simulink model "TDOF_simulink_v2"  (R2026a)
settings: Solver=VariableStepAuto  StopTime=180  MaxStep=0.001
InitFcn:
  | model_path = fileparts(get_param(bdroot, 'FileName'));
  | parent_path = fileparts(model_path);
  | run(fullfile(parent_path, 'scripts', 'NewInitFcn.m'));
undefined symbols (not defined in the file): chute, data, envP, launch, r
libraries: simulink x5
settings Model: Creator=awint  LastModifiedBy=benjaminbrobst

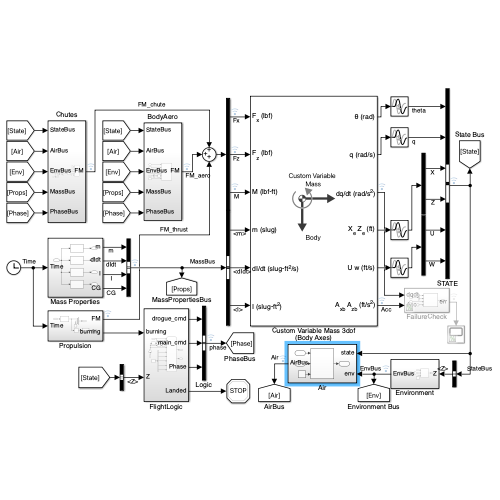
[thumbnail: Simulink's stored preview of the top-level diagram]
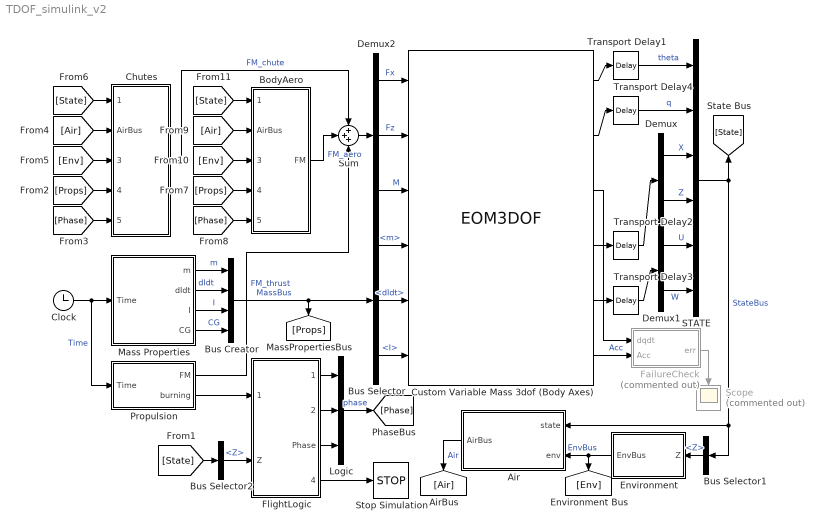
== system TDOF_simulink_v2 ==
  Air : Subsystem
  BodyAero : Subsystem
  Bus Creator : BusCreator  Inputs=4
  Bus Selector : BusSelector  OutputSignals=m,dIdt,I
  Bus Selector1 : BusSelector  OutputSignals=Z
  Bus Selector2 : BusSelector  OutputSignals=Z
  Chutes : Subsystem
  Clock : Clock
  Custom Variable Mass 3dof (Body Axes) : EOM3DOF  units=English (velocity in ft/s)  mtype=Custom Variable  v_ini=0  theta_ini=launch.theta0  g=32.174
  Demux : Demux  Outputs=2
  Demux1 : Demux  Outputs=2
  Demux2 : Demux  Outputs=3
  Environment : Subsystem
  FailureCheck : Subsystem  Commented=on
  FlightLogic : Subsystem
  Logic : BusCreator  Inputs=3
  Mass Properties : Subsystem
  Propulsion : Subsystem
  STATE : BusCreator  Inputs=6
  Scope : Scope  Commented=on
  Stop Simulation : Stop
  Sum : Sum  Inputs=+++
  Transport Delay1 : TransportDelay  DelayTime=0.001  InitialOutput=launch.theta0
  Transport Delay2 : TransportDelay  DelayTime=0.001
  Transport Delay3 : TransportDelay  DelayTime=0.001
  Transport Delay4 : TransportDelay  DelayTime=0.001
  wires:
  Custom Variable Mass 3dof (Body Axes)/1 -> Transport Delay1/1
  Custom Variable Mass 3dof (Body Axes)/2 -> Transport Delay4/1
  STATE/1 -> [State], Bus Selector1/1, Air/1(state)  "StateBus"
  Demux2/1 -> Custom Variable Mass 3dof (Body Axes)/1  "Fx"
  Demux2/2 -> Custom Variable Mass 3dof (Body Axes)/2  "Fz"
  Demux2/3 -> Custom Variable Mass 3dof (Body Axes)/3  "M"
  Clock/1 -> Mass Properties/1(Time), Propulsion/1(Time)  "Time"
  Bus Selector/1 -> Custom Variable Mass 3dof (Body Axes)/4  "<m>"
  Bus Selector/2 -> Custom Variable Mass 3dof (Body Axes)/5  "<dIdt>"
  Bus Selector/3 -> Custom Variable Mass 3dof (Body Axes)/6  "<I>"
  Propulsion/1(FM) -> Sum/3  "FM_thrust"
  Bus Creator/1 -> Bus Selector/1, [Props]  "MassBus"
  Bus Selector1/1 -> Environment/1(Z)  "<Z>"
  Environment/1(EnvBus) -> [Env], Air/2(env)  "EnvBus"
  Air/1(AirBus) -> [Air]  "Air"
  Propulsion/2(burning) -> FlightLogic/1(burning)
  FlightLogic/4(Landed) -> Stop Simulation/1
  [State] -> Bus Selector2/1
  Bus Selector2/1 -> FlightLogic/2(Z)  "<Z>"
  FlightLogic/3(Phase) -> Logic/3
  FlightLogic/2(main_cmd) -> Logic/2
  FlightLogic/1(drogue_cmd) -> Logic/1
  Logic/1 -> [Phase]  "phase"
  [Props] -> Chutes/4(MassBus)
  [Phase] -> Chutes/5(PhaseBus)
  [State] -> Chutes/1(StateBus)
  [Air] -> Chutes/2(AirBus)
  [Env] -> Chutes/3(EnvBus)
  [State] -> BodyAero/1(StateBus)
  [Air] -> BodyAero/2(AirBus)
  [Env] -> BodyAero/3(EnvBus)
  [Props] -> BodyAero/4(MassBus)
  [Phase] -> BodyAero/5(PhaseBus)
  Chutes/1(FM) -> Sum/1  "FM_chute"
  BodyAero/1(FM) -> Sum/2  "FM_aero"
  Mass Properties/1(m) -> Bus Creator/1  "m"
  Mass Properties/2(dIdt) -> Bus Creator/2  "dIdt"
  Mass Properties/3(I) -> Bus Creator/3  "I"
  Mass Properties/4(CG) -> Bus Creator/4  "CG"
  Transport Delay1/1 -> STATE/1  "theta"
  Transport Delay4/1 -> STATE/2  "q"
  Demux/1 -> STATE/3  "X"
  Demux/2 -> STATE/4  "Z"
  Demux1/1 -> STATE/5  "U"
  Demux1/2 -> STATE/6  "W"
  Custom Variable Mass 3dof (Body Axes)/6 -> FailureCheck/2(Acc)  "Acc"
  Custom Variable Mass 3dof (Body Axes)/4 -> Transport Delay2/1
  Custom Variable Mass 3dof (Body Axes)/5 -> Transport Delay3/1
  Transport Delay3/1 -> Demux1/1
  Transport Delay2/1 -> Demux/1
  Sum/1 -> Demux2/1
  Custom Variable Mass 3dof (Body Axes)/3 -> FailureCheck/1(dqdt)
  FailureCheck/1(err) -> Scope/1

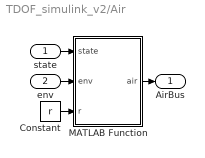
== system TDOF_simulink_v2/Air ==
  state : Inport  OutDataTypeStr=Bus: StateBus
  env : Inport  Port=2  OutDataTypeStr=Bus: EnvBus
  Constant : Constant  Value=r  OutDataTypeStr=Bus: slBus1
  MATLAB Function : MATLAB Function  TreatAsAtomicUnit=on
  AirBus : Outport  OutDataTypeStr=Bus: AirBus
  wires:
  env/1 -> MATLAB Function/2(env)
  state/1 -> MATLAB Function/1(state)
  Constant/1 -> MATLAB Function/3(r)
  MATLAB Function/1(air) -> AirBus/1

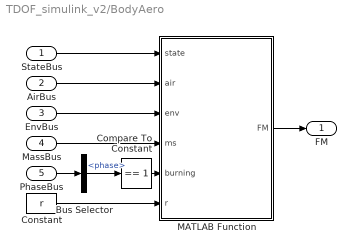
== system TDOF_simulink_v2/BodyAero ==
  StateBus : Inport  OutDataTypeStr=Bus: StateBus
  AirBus : Inport  Port=2  OutDataTypeStr=Bus: AirBus
  EnvBus : Inport  Port=3  OutDataTypeStr=Bus: EnvBus
  MassBus : Inport  Port=4  OutDataTypeStr=Bus: MassBus
  PhaseBus : Inport  Port=5  OutDataTypeStr=Bus: PhaseBus
  Bus Selector : BusSelector  OutputSignals=phase
  Compare To Constant : simulink/Logic and Bit Operations/Compare To Constant  relop===  const=1  OutDataTypeStr=boolean
  Constant : Constant  Value=r  OutDataTypeStr=Bus: slBus1
  MATLAB Function : MATLAB Function  TreatAsAtomicUnit=on
  FM : Outport
  wires:
  MATLAB Function/1(FM) -> FM/1
  StateBus/1 -> MATLAB Function/1(state)
  AirBus/1 -> MATLAB Function/2(air)
  EnvBus/1 -> MATLAB Function/3(env)
  MassBus/1 -> MATLAB Function/4(ms)
  PhaseBus/1 -> Bus Selector/1
  Bus Selector/1 -> Compare To Constant/1  "<phase>"
  Compare To Constant/1 -> MATLAB Function/5(burning)
  Constant/1 -> MATLAB Function/6(r)

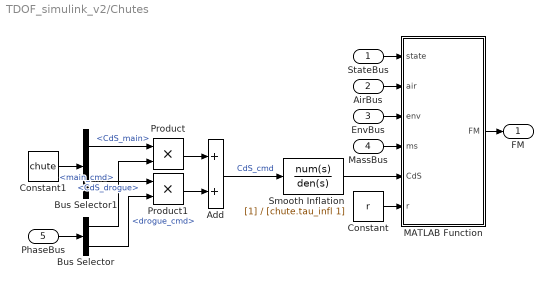
== system TDOF_simulink_v2/Chutes ==
  StateBus : Inport  OutDataTypeStr=Bus: StateBus
  AirBus : Inport  Port=2  OutDataTypeStr=Bus: AirBus
  EnvBus : Inport  Port=3  OutDataTypeStr=Bus: EnvBus
  MassBus : Inport  Port=4  OutDataTypeStr=Bus: MassBus
  PhaseBus : Inport  Port=5  OutDataTypeStr=Bus: PhaseBus
  Add : Sum
  Bus Selector : BusSelector  OutputSignals=main_cmd,drogue_cmd
  Bus Selector1 : BusSelector  OutputSignals=CdS_main,CdS_drogue
  Constant : Constant  Value=r  OutDataTypeStr=Bus: slBus1
  Constant1 : Constant  Value=chute  OutDataTypeStr=Bus: slBus3
  MATLAB Function : MATLAB Function  TreatAsAtomicUnit=on
  Product : Product
  Product1 : Product
  Smooth Inflation : TransferFcn  Denominator=[chute.tau_infl 1]
  FM : Outport
  wires:
  StateBus/1 -> MATLAB Function/1(state)
  AirBus/1 -> MATLAB Function/2(air)
  MATLAB Function/1(FM) -> FM/1
  EnvBus/1 -> MATLAB Function/3(env)
  MassBus/1 -> MATLAB Function/4(ms)
  Constant/1 -> MATLAB Function/6(r)
  PhaseBus/1 -> Bus Selector/1
  Bus Selector/1 -> Product/2  "<main_cmd>"
  Bus Selector/2 -> Product1/2  "<drogue_cmd>"
  Constant1/1 -> Bus Selector1/1
  Bus Selector1/1 -> Product/1  "<CdS_main>"
  Bus Selector1/2 -> Product1/1  "<CdS_drogue>"
  Product/1 -> Add/1
  Product1/1 -> Add/2
  Add/1 -> Smooth Inflation/1  "CdS_cmd"
  Smooth Inflation/1 -> MATLAB Function/5(CdS)

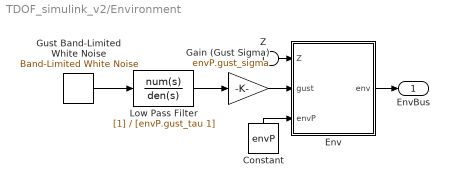
== system TDOF_simulink_v2/Environment ==
  Z : Inport
  Constant : Constant  Value=envP  OutDataTypeStr=Bus: slBus2
  Env : MATLAB Function  TreatAsAtomicUnit=on
  Gain (Gust Sigma) : Gain  Gain=envP.gust_sigma
  Gust Band-Limited White Noise : simulink/Sources/Band-Limited White Noise  Cov=1  Ts=0.1  seed=envP.gust_seed
  Low Pass Filter : TransferFcn  Denominator=[envP.gust_tau 1]
  EnvBus : Outport  OutDataTypeStr=Bus: EnvBus
  wires:
  Env/1(env) -> EnvBus/1
  Z/1 -> Env/1(Z)
  Gain (Gust Sigma)/1 -> Env/2(gust)
  Constant/1 -> Env/3(envP)
  Gust Band-Limited White Noise/1 -> Low Pass Filter/1
  Low Pass Filter/1 -> Gain (Gust Sigma)/1

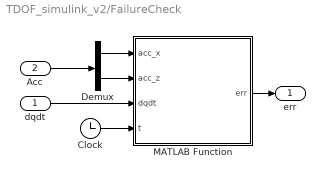
== system TDOF_simulink_v2/FailureCheck ==
  dqdt : Inport
  Acc : Inport  Port=2
  Clock : Clock
  Demux : Demux  Outputs=2
  MATLAB Function : MATLAB Function  TreatAsAtomicUnit=on
  err : Outport
  wires:
  Acc/1 -> Demux/1
  dqdt/1 -> MATLAB Function/3(dqdt)
  Demux/2 -> MATLAB Function/2(acc_z)
  Demux/1 -> MATLAB Function/1(acc_x)
  Clock/1 -> MATLAB Function/4(t)
  MATLAB Function/1(err) -> err/1

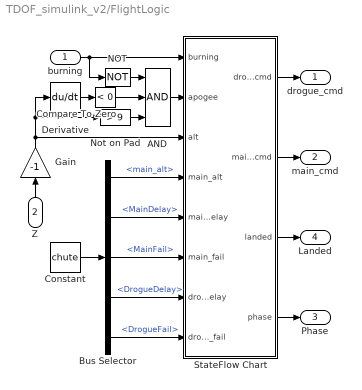
== system TDOF_simulink_v2/FlightLogic ==
  burning : Inport
  Z : Inport  Port=2
  AND : Logic  Inputs=3  AllPortsSameDT=off  OutDataTypeStr=boolean
  Bus Selector : BusSelector  OutputSignals=main_alt,MainDelay,MainFail,DrogueDelay,DrogueFail
  Compare To Zero : simulink/Logic and Bit Operations/Compare To Zero  relop=<  OutDataTypeStr=boolean  ZeroCross=off
  Constant : Constant  Value=chute  OutDataTypeStr=Bus: slBus3
  Derivative : Derivative
  Gain : Gain  Gain=-1
  NOT : Logic  Operator=NOT  AllPortsSameDT=off  OutDataTypeStr=boolean
  Not on Pad : simulink/Logic and Bit Operations/Compare To Constant  relop=>  const=9  OutDataTypeStr=boolean
  StateFlow Chart : Stateflow chart  TreatAsAtomicUnit=on
  drogue_cmd : Outport
  main_cmd : Outport  Port=2
  Phase : Outport  Port=3
  Landed : Outport  Port=4
  wires:
  Z/1 -> Gain/1
  burning/1 -> StateFlow Chart/1(burning), NOT/1
  StateFlow Chart/1(drogue_cmd) -> drogue_cmd/1
  StateFlow Chart/2(main_cmd) -> main_cmd/1
  StateFlow Chart/3(landed) -> Landed/1
  StateFlow Chart/4(phase) -> Phase/1
  Constant/1 -> Bus Selector/1
  Bus Selector/1 -> StateFlow Chart/4(main_alt)  "<main_alt>"
  Bus Selector/5 -> StateFlow Chart/8(drogue_fail)  "<DrogueFail>"
  Bus Selector/2 -> StateFlow Chart/5(main_delay)  "<MainDelay>"
  Bus Selector/3 -> StateFlow Chart/6(main_fail)  "<MainFail>"
  Bus Selector/4 -> StateFlow Chart/7(drogue_delay)  "<DrogueDelay>"
  AND/1 -> StateFlow Chart/2(apogee)
  NOT/1 -> AND/1
  Compare To Zero/1 -> AND/2
  Derivative/1 -> Compare To Zero/1
  Not on Pad/1 -> AND/3
  Gain/1 -> Derivative/1, Not on Pad/1, StateFlow Chart/3(alt)

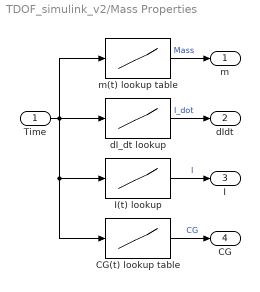
== system TDOF_simulink_v2/Mass Properties ==
  Time : Inport
  CG(t) lookup table : Lookup_n-D  NumberOfTableDimensions=1  BreakpointsForDimension1=data.time_vec  Table=data.CG_vec  ExtrapMethod=Clip  UseLastTableValue=on  InternalRulePriority=Speed  RndMeth=Simplest
  I(t) lookup : Lookup_n-D  NumberOfTableDimensions=1  BreakpointsForDimension1=data.time_vec  Table=data.I_vec  ExtrapMethod=Clip  UseLastTableValue=on  InternalRulePriority=Speed  RndMeth=Simplest
  dI_dt lookup : Lookup_n-D  NumberOfTableDimensions=1  BreakpointsForDimension1=data.time_vec(1:end-1)  Table=data.dI_dt_vec  ExtrapMethod=Clip  UseLastTableValue=on  InternalRulePriority=Speed  RndMeth=Simplest
  m(t) lookup table : Lookup_n-D  NumberOfTableDimensions=1  BreakpointsForDimension1=data.time_vec  Table=data.tot_mass_vec  ExtrapMethod=Clip  UseLastTableValue=on  InternalRulePriority=Speed  RndMeth=Simplest
  m : Outport
  dIdt : Outport  Port=2
  I : Outport  Port=3
  CG : Outport  Port=4
  wires:
  I(t) lookup/1 -> I/1  "I"
  Time/1 -> CG(t) lookup table/1, I(t) lookup/1, dI_dt lookup/1, m(t) lookup table/1
  dI_dt lookup/1 -> dIdt/1  "I_dot"
  m(t) lookup table/1 -> m/1  "Mass"
  CG(t) lookup table/1 -> CG/1  "CG"

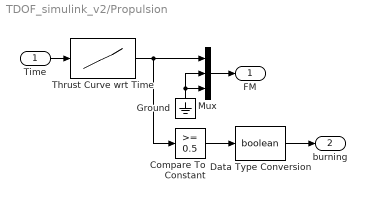
== system TDOF_simulink_v2/Propulsion ==
  Time : Inport
  Compare To Constant : simulink/Logic and Bit Operations/Compare To Constant  relop=>=  const=0.5  OutDataTypeStr=boolean
  Data Type Conversion : DataTypeConversion  OutDataTypeStr=boolean  SaturateOnIntegerOverflow=off  RndMeth=Floor
  Ground : Ground
  Mux : Mux  Inputs=3
  Thrust Curve wrt Time : Lookup_n-D  NumberOfTableDimensions=1  BreakpointsForDimension1=data.time_vec  Table=data.thrust_vec  ExtrapMethod=Clip  UseLastTableValue=on  InternalRulePriority=Speed  RndMeth=Simplest
  FM : Outport
  burning : Outport  Port=2
  wires:
  Time/1 -> Thrust Curve wrt Time/1
  Mux/1 -> FM/1
  Ground/1 -> Mux/3, Mux/2
  Thrust Curve wrt Time/1 -> Compare To Constant/1, Mux/1
  Compare To Constant/1 -> Data Type Conversion/1
  Data Type Conversion/1 -> burning/1

== matlab function TDOF_simulink_v2/Environment/Env ==
  data: Z input; env output Bus: EnvBus; gust input; envP input
function env = Environment_blk(Z, gust,envP)
% Edit the function Environment.m in MATLAB proper for easier commits.
env = Environment(Z,gust,envP);
end

== matlab function TDOF_simulink_v2/BodyAero/MATLAB Function ==
  data: state input Bus: StateBus; FM output; air input Bus: AirBus; env input Bus: EnvBus; ms input Bus: MassBus; burning input boolean; r input Bus: slBus1
function FM = BodyAero_blk(state, air, env, ms, burning, r)
% From the current state, air, environment, mass properties, phase, and
% fixed rocket characteristics, determine the forces and moments on the
% body.
% To edit this function, go to BodyAero.m. This is done for a better commit
% structure.
FM = BodyAero(state, air, env, ms, burning, r);
end

== matlab function TDOF_simulink_v2/FailureCheck/MATLAB Function ==
  data: acc_x input; err output; acc_z input; dqdt input; t input
function err = failureMode_blk(acc_x,acc_z,dqdt,t)
% failureMode_blk -- runs failureMode.m script in /scripts/functions.
% If linear or angular acceleration is too much, yield a warning/error
% string.
err = failureMode(acc_x,acc_z,dqdt,t);

== matlab function TDOF_simulink_v2/Chutes/MATLAB Function ==
  data: state input Bus: StateBus; FM output; air input Bus: AirBus; env input Bus: EnvBus; ms input Bus: MassBus; CdS input; r input Bus: slBus1
function FM = Chute_blk(state, air, env, ms, CdS, r)
% Returns the forces and moments associated with drogue or drogue and main
% deployment.
% To edit this function, see the file Chute.m and edit there for better
% commit structuring.
FM = Chute(state, air, env, ms, CdS, r);
end

== matlab function TDOF_simulink_v2/Air/MATLAB Function ==
  data: state input Bus: StateBus; env input Bus: EnvBus; air output Bus: AirBus; r input Bus: slBus1
function air = AirData_blk(state, env, r)
% Converts environmental data into air data relevant and relative to the
% rocket's current frame. Also gives dynamic pressure, mach number, and
% angle of attack (alpha).
% To edit this function, goto the actual AirData.m script (for better
% GitHub commits).
air = AirData(env,state,r);
end

== stateflow chart TDOF_simulink_v2/FlightLogic/StateFlow Chart ==
  settings: updateMethod=DISCRETE  sampleTime=0.01
  state FlightPhase [parallel]
    settings: executionOrder=1
    state Pad
      en: phase=0; drogue_cmd=0; main_cmd=0; landed=0;
    state Boost
      en: phase=1;
    state Coast
      en: phase=2;
    state Drogue
      en: phase=3;
    state Landed
      en: phase=6; landed=1;
    state MainDelay
      en: phase=4;
    state Main
      en: phase=5;
    (default) -> Pad
    Pad -> Boost : [burning]
    Boost -> Landed [order 2] : [alt <= -5]
    Boost -> Coast [order 1] : [~burning]
    Coast -> Landed [order 2] : [alt <= 0]
    Coast -> Drogue [order 1] : [apogee]
    Drogue -> Landed [order 2] : [alt <= 0]
    Drogue -> MainDelay [order 1] : [alt < main_alt]
    Main -> Landed : [alt <= 0]
    MainDelay -> Landed [order 2] : [alt <= 0]
    MainDelay -> Main [order 1] : after(main_delay, sec)
  state DrogueLogic [parallel]
    settings: executionOrder=2
    state Stowed
    state Pending
    state Failed
      en: drogue_cmd=0;
    state Deployed
      en: drogue_cmd=1;
    (default) -> DrogueLogic.Stowed
    DrogueLogic.Stowed -> Pending [order 1] : [in(FlightPhase.Drogue) && ~drogue_fail]
    DrogueLogic.Stowed -> DrogueLogic.Failed [order 2] : [in(FlightPhase.Drogue) && drogue_fail]
    Pending -> DrogueLogic.Deployed : after(drogue_delay, sec)
  state MainLogic [parallel]
    settings: executionOrder=3
    state Stowed
    state Failed
      en: main_cmd=0;
    state Deployed
      en: main_cmd=1;
    (default) -> MainLogic.Stowed
    MainLogic.Stowed -> MainLogic.Deployed [order 2] : [in(FlightPhase.Main) && ~main_fail]
    MainLogic.Stowed -> MainLogic.Failed [order 1] : [in(FlightPhase.Main) && main_fail]
  data: burning input boolean; apogee input boolean; alt input double; drogue_cmd output double; main_cmd output double; landed output double; phase output double; main_alt input double; main_delay input; main_fail input; drogue_delay input; drogue_fail input
